simulink model "heli_q8_Lab3_primary"  (R2020b)
settings: Solver=ode1  StartTime=0.0  StopTime=inf  FixedStep=0.002  RelTol=1e-3  EnableMultiTasking=on
PostLoadFcn:
  | qc_set_target_type(getConfigSet(bdroot, 'QUARC Default Target Configuration'));
values from neighbouring files (symbols this model uses):
  A_lqr = [0, 1, 0, 0, 0 ... (first row only)    [init_heli_Lab3_extra.m]    (also in init_heli_Lab3_primary.m)
  B = [0 0; 0 K1; K2 0; 0 0; 0 0]    [init_heli_Lab3_extra.m]    (also in init_heli_Lab3_primary.m)
  C_lqr = [0 0 0 0 0 ... (first row only)    [init_heli_Lab3_extra.m]    (also in init_heli_Lab3_primary.m = [1 0 0 0 0)
  F = [0 0; 0 0]    [init_heli_Lab3_extra.m]    (also in init_heli_Lab3_primary.m = [1 0; 1 0])
  Joystick_gain_x = 1    [init_heli_Lab3_extra.m]    (also in init_heli_Lab3_primary.m)
  Joystick_gain_y = -1    [init_heli_Lab3_extra.m]    (also in init_heli_Lab3_primary.m)
  K_pd = -(lambda_1 + lambda_2)/K1    [init_heli_Lab3_extra.m]    (also in init_heli_Lab3_primary.m)
  K_pp = (lambda_1*lambda_2)/K1    [init_heli_Lab3_extra.m]    (also in init_heli_Lab3_primary.m)
  L = place(A_lqr', C_lqr', p).'    [init_heli_Lab3_extra.m]    (also in init_heli_Lab3_primary.m)
undefined symbols (not defined in the file or in its folder): HIL, K, qc_get_step_size
libraries: quarc_library x9
settings Model: SimulationMode=external  ExtModeTrigDuration=5000  Creator=Rchan  LastModifiedBy=pederaho
settings SolverCC: PositivePriorityOrder=on
settings DataIOCC: LimitDataPoints=on  SaveFormat=Array  SignalLoggingSaveFormat=ModelDataLogs  ReturnWorkspaceOutputs=off
settings OptimizationCC: ExpressionDepthLimit=2147483647  InitFltsAndDblsToZero=on  LifeSpan=inf
settings DebuggingCC: SaveWithParameterizedLinksMsg=none  UnderspecifiedInitializationDetection=Classic  MergeDetectMultiDrivingBlocksExec=none  SolverPrmCheckMsg=warning  MultiTaskDSMMsg=warning  MultiTaskCondExecSysMsg=none  FcnCallInpInsideContextMsg=warning  AllowSymbolicDim=off  StateNameClashWarn=warning  SFUnexpectedBacktrackingDiag=warning  SFNoUnconditionalDefaultTransitionDiag=warning  SFExecutionAtInitializationDiag=none  ArithmeticOperatorsInVariantConditions=warning
settings HardwareCC: ProdBitPerPointer=32  ProdBitPerSizeT=32  ProdBitPerPtrDiffT=32  ProdLargestAtomicFloat=None  ProdIntDivRoundTo=Undefined  ProdEndianess=Unspecified  ProdWordSize=32  ProdHWDeviceType=32-bit Generic
settings ModelReferenceCC: PropagateSignalLabelsOutOfModel=off
settings SFSimCC: SimUseLocalCustomCode=off  CustomCodeUndefinedFunction=UseInterfaceOnly
settings RTWCC: Description=QUARC Win64 Target  SystemTargetFile=quarc_win64.tlc  TemplateMakefile=quarc_default_tmf  RTWUseLocalCustomCode=off
settings CodeAppCC: StateflowObjectComments=on
settings GRTTargetCC: TargetLangStandard=C89/C90 (ANSI)  ParMdlRefBuildCompliant=off  CompOptLevelCompliant=off  CombineOutputUpdateFcns=off  MatFileLogging=off  GRTInterface=on  UseToolchainInfoCompliant=off  ExtMode=on  ExtModeMexFile=quarc_comm
settings ConfigComp: CovMetricSettings=dw  CovSaveCumulativeToWorkspaceVar=on  CovSaveSingleToWorkspaceVar=on  CovExternalEMLEnable=off  CovSFcnEnable=off

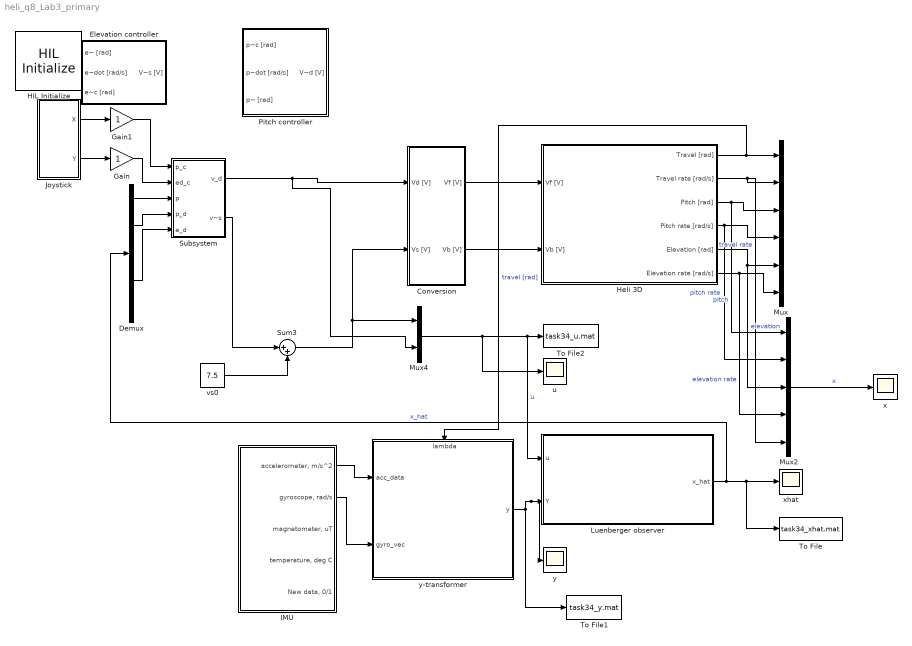
== system heli_q8_Lab3_primary ==
  Conversion : Subsystem
  Demux : Demux  Outputs=5
  Elevation controller : Subsystem
  Gain : Gain
  Gain1 : Gain
  HIL Initialize : quarc_library/Data Acquisition/Generic/Configuration/HIL Initialize  Priority=-99  object_name=HIL-1  board_type=q8_usb  board_number=0  board_options=update_rate=normal;decimation=1  exclusive=off  active=off  hardware_clocks=[0:2]  clock_modes=[]  initial_clock_frequencies=[]  set_clock_params_at_start=off  set_clock_params_at_switch_in=off  set_clock_frequencies_at_start=off  set_clock_frequencies_at_switch_in=off  analog_input_channels=[0:7]  analog_input_configurations=[]  analog_input_maximums=10  analog_input_minimums=-10  set_analog_input_params_at_start=on  set_analog_input_params_at_switch_in=off  analog_output_channels=[0:7]  analog_output_maximums=10  analog_output_minimums=-10  initial_analog_outputs=[0]  final_analog_outputs=[0]  watchdog_analog_outputs=0  set_analog_output_params_at_start=on  set_analog_output_params_at_switch_in=off  set_analog_outputs_at_start=on  set_analog_outputs_at_switch_in=off  set_analog_outputs_at_terminate=on  set_analog_outputs_at_switch_out=off  set_analog_outputs_on_watchdog=off  digital_input_channels=[]  digital_output_channels=[]  digital_output_configuration=[]  initial_digital_outputs=[1]  final_digital_outputs=[1]  watchdog_digital_outputs=[1]  set_digital_output_params_at_start=off  set_digital_output_params_at_switch_in=off  set_digital_outputs_at_start=on  set_digital_outputs_at_switch_in=off  set_digital_outputs_at_terminate=on  set_digital_outputs_at_switch_out=off  set_digital_outputs_on_watchdog=off  encoder_channels=[0:7]  quadrature=[4]  encoder_filter_frequency=[]  initial_encoder_counts=[0]  set_encoder_params_at_start=on  set_encoder_params_at_switch_in=off  set_encoder_counts_at_start=on  set_encoder_counts_at_switch_in=off  pwm_channels=[0:7]  pwm_modes=0  pwm_frequency=99.532799999999995e6/4095  pwm_configuration=[0]  pwm_alignment=[0]  pwm_polarity=[1]  pwm_leading_deadband=[0]  pwm_trailing_deadband=[0]  initial_pwm_outputs=[0]  final_pwm_outputs=[0]  watchdog_pwm_outputs=[0]  set_pwm_params_at_start=on  set_pwm_params_at_switch_in=off  set_pwm_outputs_at_start=on  set_pwm_outputs_at_switch_in=off  set_pwm_outputs_at_terminate=on  set_pwm_outputs_at_switch_out=off  set_pwm_outputs_on_watchdog=off  other_output_channels=[]  initial_other_outputs=[]  final_other_outputs=[]  watchdog_other_outputs=[]  set_other_outputs_at_start=off  set_other_outputs_at_switch_in=off  set_other_outputs_at_terminate=off  set_other_outputs_at_switch_out=off  set_other_outputs_on_watchdog=off
  Heli 3D : Subsystem
  IMU : Subsystem
  Joystick : Subsystem
  Luenberger observer : Subsystem
  Mux : Mux  Inputs=6
  Mux2 : Mux  Inputs=5
  Mux4 : Mux  Inputs=2
  Pitch controller : Subsystem
  Subsystem : Subsystem
  Sum3 : Sum  Inputs=|++
  To File : ToFile  Filename=task34_xhat.mat
  To File1 : ToFile  Filename=task34_y.mat
  To File2 : ToFile  Filename=task34_u.mat
  u : Scope
  vs0 : Constant  Value=7.5
  x : Scope
  xhat : Scope
  y : Scope
  y-transformer : Subsystem
      settings: PortSchema="{\"entries\":[{\"content\":{\"sides\":[{\"content\":{\"connectorIds\":[\"In1\",\"In2\"]},\"type\":\"ConnectorPlacement.EquallySpacedRectSide\",\"uuid\":\"7fe3842c-12da-4414-9d6c-fe9db8df7207\"},{\"content\":{\"connectorIds\":[\"Out1\"],\"side\":\"RIGHT\"},\"type\":\"ConnectorPlacement.EquallySpacedRectSide\",\"uuid\":\"81ab8372-6ad3-4160-a082-397e448f1dbf\"},{\"content\":{\"connectorIds\":[\"In3\"],\"side\":\"TOP\"},\"type\":\"ConnectorPlacement.EquallySpacedRectSide\",\"uuid\":\"eccdd19c-8bf4-44ad-b1cc-041d97ac8cb4\"},{\"content\":{\"connectorIds\":[],\"side\":\"HIDDEN\"},\"type\":\"ConnectorPlacement.EquallySpacedRectSide\",\"uuid\":\"e5e0ccf8-496d-4101-9f4c-362465ae7577\"}]},\"type\":\"ConnectorPlacement.EquallySpacedConnector\",\"uuid\":\"e1e81078-5ff0-43da-8bd4-b4064180551e\"}],\"packageUris\":[\"http://schema.mathworks.com/mf0/Connector/R2020b\"],\"version\":\"1.0\"}"
  wires:
  Mux2/1 -> x/1  "x"
  IMU/1("accelerometer, m/s^2") -> y-transformer/1(acc_data)
  Gain1/1 -> Subsystem/1(p_c)
  vs0/1 -> Sum3/2
  Subsystem/1(v_d) -> Mux4/2, Conversion/1(Vd [V])
  Demux/1 -> Subsystem/3(p)
  Sum3/1 -> Mux4/1, Conversion/2(Vs [V])
  Demux/2 -> Subsystem/4(p_d)
  Demux/4 -> Subsystem/5(e_d)
  Subsystem/2(v~s) -> Sum3/1
  IMU/2("gyroscope, rad/s") -> y-transformer/2(gyro_vec)
  Gain/1 -> Subsystem/2(ed_c)
  Joystick/2(Y) -> Gain/1
  Heli 3D/3(Pitch [rad]) -> Mux/3, Mux2/1  "pitch"
  Joystick/1(X) -> Gain1/1
  Heli 3D/1(Travel [rad]) -> Mux/1, y-transformer/3(lambda)  "travel [rad]"
  Conversion/1(Vf [V]) -> Heli 3D/1(Vf [V])
  Heli 3D/5(Elevation [rad]) -> Mux/5, Mux2/3  "elevation"
  Heli 3D/6(Elevation rate [rad/s]) -> Mux/6, Mux2/4  "elevation rate"
  Conversion/2(Vb [V]) -> Heli 3D/2(Vb [V])
  Luenberger observer/1(x_hat) -> xhat/1, To File/1, Demux/1  "x_hat"
  y-transformer/1(y) -> y/1, Luenberger observer/2(Y), To File1/1
  Mux4/1 -> Luenberger observer/1(u), To File2/1, u/1  "u"
  Heli 3D/2(Travel rate [rad/s]) -> Mux/2, Mux2/5  "travel rate"
  Heli 3D/4(Pitch rate [rad/s]) -> Mux/4, Mux2/2  "pitch rate"

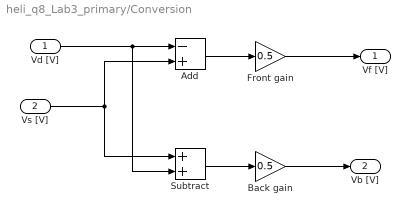
== system heli_q8_Lab3_primary/Conversion ==
  Vd [V] : Inport
  Vs [V] : Inport  Port=2
  Add : Sum  Inputs=-+
  Back gain : Gain  Gain=0.5
  Front gain : Gain  Gain=0.5
  Subtract : Sum
  Vf [V] : Outport
  Vb [V] : Outport  Port=2
  wires:
  Vd [V]/1 -> Subtract/2, Add/1
  Vs [V]/1 -> Subtract/1, Add/2
  Subtract/1 -> Back gain/1
  Back gain/1 -> Vb [V]/1
  Add/1 -> Front gain/1
  Front gain/1 -> Vf [V]/1

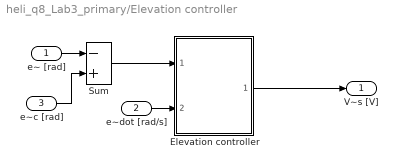
== system heli_q8_Lab3_primary/Elevation controller ==
  e~ [rad] : Inport
  e~dot [rad/s] : Inport  Port=2
  e~c [rad] : Inport  Port=3
  Elevation controller : Subsystem
  Sum : Sum  Inputs=-+  InputSameDT=on  SaturateOnIntegerOverflow=on  OutDataTypeStr=Inherit: Same as first input
  V~s [V] : Outport  InitialOutput=0
  wires:
  Sum/1 -> Elevation controller/1(e~ [rad])
  Elevation controller/1(V~_s [V]) -> V~s [V]/1
  e~ [rad]/1 -> Sum/1
  e~dot [rad/s]/1 -> Elevation controller/2(e~_dot [rad/s])
  e~c [rad]/1 -> Sum/2

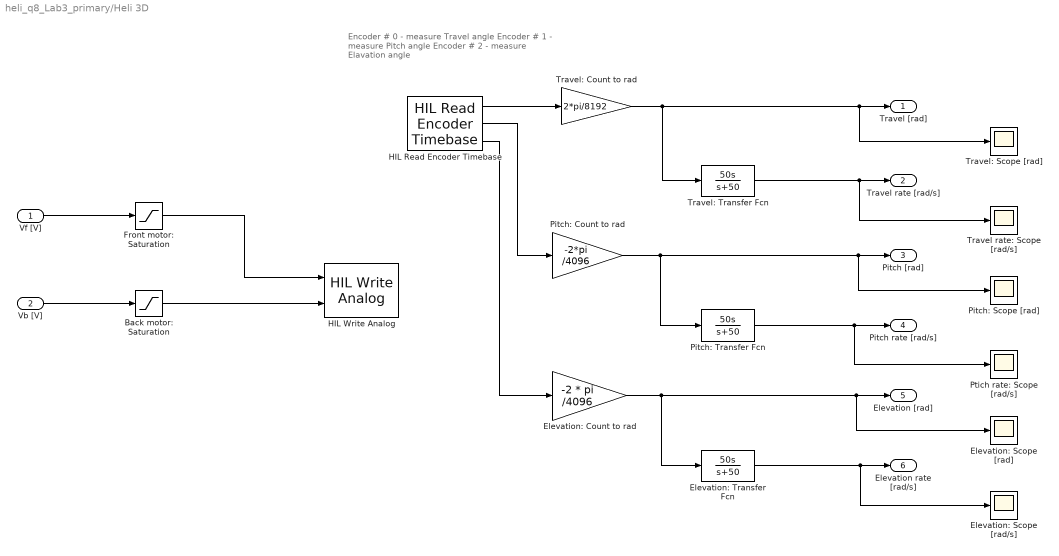
== system heli_q8_Lab3_primary/Heli 3D ==
  note: Encoder # 0 - measure Travel angle
      | Encoder # 1 - measure Pitch angle
      | Encoder # 2 - measure Elavation angle
  Vf [V] : Inport
  Vb [V] : Inport  Port=2
  Back motor: Saturation : Saturate  UpperLimit=5  LowerLimit=-5
  Elevation: Count to rad : Gain  Gain=-2 * pi /4096
  Elevation: Scope [rad/s] : Scope
  Elevation: Scope [rad] : Scope
  Elevation: Transfer Fcn : TransferFcn  Numerator=[50 0]  Denominator=[1 50]
  Front motor: Saturation : Saturate  UpperLimit=5  LowerLimit=-5
  HIL Read Encoder Timebase : quarc_library/Data Acquisition/Generic/Timebases/HIL Read Encoder Timebase  object_name=HIL-1  clock=0  channels=[0:2]  active=on  vector_output=off  data_type_mode=Inherit via back propagation  data_type=double  overflow_mode=Error on overflow  samples_in_buffer=max(ceil(1/qc_get_step_size), 1)
  HIL Write Analog : quarc_library/Data Acquisition/Generic/Immediate I//O/HIL Write Analog  object_name=HIL-1  channels=[0:1]  sample_time=-1  active=off  vector_input=off
  Pitch: Count to rad : Gain  Gain=-2*pi /4096
  Pitch: Scope [rad] : Scope
  Pitch: Transfer Fcn : TransferFcn  Numerator=[50 0]  Denominator=[1 50]
  Ptich rate: Scope [rad/s] : Scope
  Travel rate: Scope [rad/s] : Scope
  Travel: Count to rad : Gain  Gain=2*pi/8192
  Travel: Scope [rad] : Scope
  Travel: Transfer Fcn : TransferFcn  Numerator=[50 0]  Denominator=[1 50]
  Travel [rad] : Outport
  Travel rate [rad/s] : Outport  Port=2
  Pitch [rad] : Outport  Port=3
  Pitch rate [rad/s] : Outport  Port=4
  Elevation [rad] : Outport  Port=5
  Elevation rate [rad/s] : Outport  Port=6
  wires:
  HIL Read Encoder Timebase/1 -> Travel: Count to rad/1
  HIL Read Encoder Timebase/2 -> Pitch: Count to rad/1
  HIL Read Encoder Timebase/3 -> Elevation: Count to rad/1
  Travel: Count to rad/1 -> Travel: Scope [rad]/1, Travel [rad]/1, Travel: Transfer Fcn/1
  Travel: Transfer Fcn/1 -> Travel rate: Scope [rad/s]/1, Travel rate [rad/s]/1
  Pitch: Count to rad/1 -> Pitch: Transfer Fcn/1, Pitch: Scope [rad]/1, Pitch [rad]/1
  Pitch: Transfer Fcn/1 -> Ptich rate: Scope [rad/s]/1, Pitch rate [rad/s]/1
  Elevation: Count to rad/1 -> Elevation: Transfer Fcn/1, Elevation: Scope [rad]/1, Elevation [rad]/1
  Elevation: Transfer Fcn/1 -> Elevation: Scope [rad/s]/1, Elevation rate [rad/s]/1
  Vf [V]/1 -> Front motor: Saturation/1
  Vb [V]/1 -> Back motor: Saturation/1
  Front motor: Saturation/1 -> HIL Write Analog/1
  Back motor: Saturation/1 -> HIL Write Analog/2

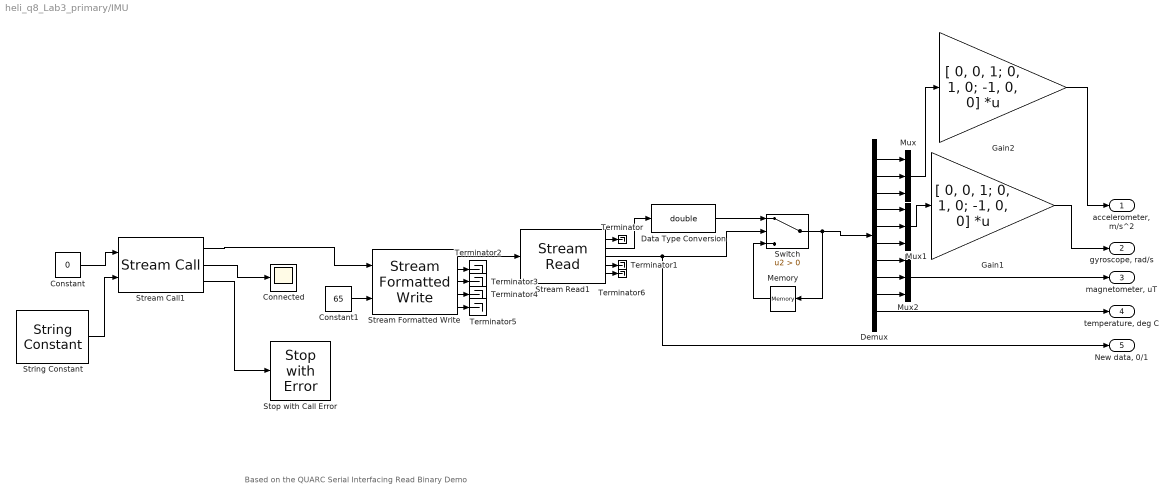
== system heli_q8_Lab3_primary/IMU ==
  note: Based on the QUARC Serial Interfacing Read Binary Demo
  Connected : Scope
  Constant : Constant  Value=0
  Constant1 : Constant  Value=65
  Data Type Conversion : DataTypeConversion  OutDataTypeStr=double
  Demux : Demux  Outputs=10
  Gain1 : Gain  Gain=[ 0, 0, 1; 0, 1, 0; -1, 0, 0]  Multiplication=Matrix(K*u) (u vector)
  Gain2 : Gain  Gain=[ 0, 0, 1; 0, 1, 0; -1, 0, 0]  Multiplication=Matrix(K*u) (u vector)
  Memory : Memory  InitialCondition=[0 0 0 0 0 0 0 0 0 0]
  Mux : Mux  Inputs=3
  Mux1 : Mux  Inputs=3
  Mux2 : Mux  Inputs=3
  Stop with Call Error : quarc_library/Sinks/Error Handling/Stop with Error  message_type=Interpret input as error code  message=Error occurred
      settings: SourceProductName=QUARC Targets
  Stream Call1 : quarc_library/Communications/Intermediate/Stream Call  uri_source=External input port  uri=serial://IMU:9?baud=115200,word=8,parity=none,stop=1,flow='none'  apply_uri_to_all_configs=on  send_buffer_size=8000  receive_buffer_size=8000  byte_order=little endian (Intel - LSB first)  sample_time=qc_get_step_size  non_blocking=on  active=off
      settings: SourceProductName=QUARC Targets
  Stream Formatted Write : quarc_library/Communications/Intermediate/Stream Formatted Write  format_string=%c\n  max_code_units=80  optimization=Minimizing latency
      settings: SourceProductName=QUARC Targets
  Stream Read1 : quarc_library/Communications/Intermediate/Stream Read  data_type=single  type_expr=BusObject  num_elements=10  receive_dims=off
      settings: SourceProductName=QUARC Targets
  String Constant : quarc_library/Strings/String Constant  string_value=qc_perform_substitutions('serial://IMU:%{PORT}?baud=115200,word=8,parity=none,stop=1')  evaluate_string=on  string_type=URI  max_length=255  sample_time=inf  variable_size=off
      settings: AttributesFormatString="\"serial://IMU:4?baud=115200,word=8,parity=none,stop=1\""  SourceProductName=QUARC Targets
  Switch : Switch  Criteria=u2 > Threshold
  Terminator{,1..6} (7 alike) : Terminator
  "accelerometer, m/s^2" : Outport
  "gyroscope, rad/s" : Outport  Port=2
  "magnetometer, uT" : Outport  Port=3
  "temperature, deg C" : Outport  Port=4
  "New data, 0/1" : Outport  Port=5
  wires:
  Switch/1 -> Memory/1, Demux/1
  Data Type Conversion/1 -> Switch/1
  Stream Read1/3 -> "New data, 0/1"/1, Switch/2
  Stream Formatted Write/1 -> Stream Read1/1
  Constant1/1 -> Stream Formatted Write/2
  Gain1/1 -> "gyroscope, rad/s"/1
  Gain2/1 -> "accelerometer, m/s^2"/1
  Stream Read1/4 -> Terminator1/1
  Demux/10 -> "temperature, deg C"/1
  Mux1/1 -> Gain1/1
  Stream Read1/2 -> Data Type Conversion/1
  Demux/7 -> Mux2/1
  Demux/8 -> Mux2/2
  Demux/9 -> Mux2/3
  Mux2/1 -> "magnetometer, uT"/1
  Demux/6 -> Mux1/3
  Demux/5 -> Mux1/2
  Demux/4 -> Mux1/1
  Mux/1 -> Gain2/1
  Demux/3 -> Mux/3
  Demux/1 -> Mux/1
  Demux/2 -> Mux/2
  Stream Read1/1 -> Terminator/1
  Stream Call1/1 -> Stream Formatted Write/1
  Constant/1 -> Stream Call1/1
  String Constant/1 -> Stream Call1/2
  Stream Call1/2 -> Connected/1
  Stream Call1/3 -> Stop with Call Error/1
  Memory/1 -> Switch/3
  Stream Formatted Write/2 -> Terminator2/1
  Stream Formatted Write/3 -> Terminator3/1
  Stream Formatted Write/4 -> Terminator4/1
  Stream Formatted Write/5 -> Terminator5/1
  Stream Read1/5 -> Terminator6/1

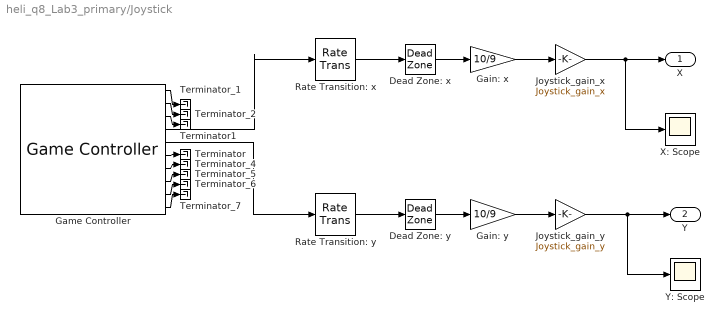
== system heli_q8_Lab3_primary/Joystick ==
  Dead Zone: x : DeadZone  LowerValue=-0.1  UpperValue=0.1  SaturateOnIntegerOverflow=on
  Dead Zone: y : DeadZone  LowerValue=-0.1  UpperValue=0.1  SaturateOnIntegerOverflow=on
  Gain: x : Gain  Gain=10/9
  Gain: y : Gain  Gain=10/9
  Game Controller : quarc_library/Devices/Peripherals/Target/Game Controller  controller=1  buffer_size=12  deadzone=[]  saturation=[]  sample_time=max(qc_get_step_size, 0.01)  auto_center=off  enabled=on
      settings: SourceProductName=QUARC Targets
  Joystick_gain_x : Gain  Gain=Joystick_gain_x
  Joystick_gain_y : Gain  Gain=Joystick_gain_y
  Rate Transition: x : RateTransition
  Rate Transition: y : RateTransition
  Terminator : Terminator
  Terminator1 : Terminator
  Terminator_{1..2,4..7} (6 alike) : Terminator
  X: Scope : Scope
  Y: Scope : Scope
  X : Outport
  Y : Outport  Port=2
  wires:
  Rate Transition: y/1 -> Dead Zone: y/1
  Rate Transition: x/1 -> Dead Zone: x/1
  Game Controller/5 -> Rate Transition: y/1
  Game Controller/4 -> Rate Transition: x/1
  Game Controller/1 -> Terminator_1/1
  Game Controller/2 -> Terminator_2/1
  Game Controller/7 -> Terminator_4/1
  Game Controller/8 -> Terminator_5/1
  Game Controller/9 -> Terminator_6/1
  Game Controller/10 -> Terminator_7/1
  Game Controller/3 -> Terminator1/1
  Game Controller/6 -> Terminator/1
  Dead Zone: x/1 -> Gain: x/1
  Dead Zone: y/1 -> Gain: y/1
  Gain: x/1 -> Joystick_gain_x/1
  Gain: y/1 -> Joystick_gain_y/1
  Joystick_gain_x/1 -> X/1, X: Scope/1
  Joystick_gain_y/1 -> Y: Scope/1, Y/1

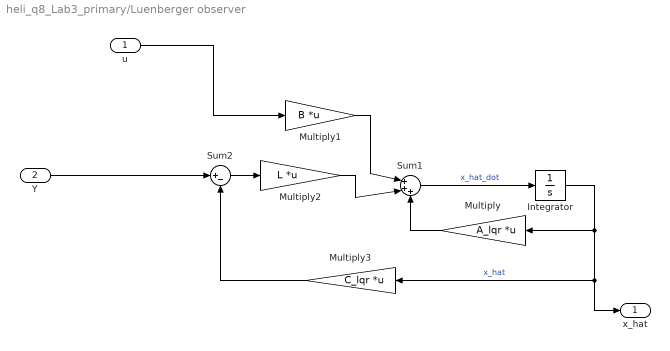
== system heli_q8_Lab3_primary/Luenberger observer ==
  u : Inport
  Y : Inport  Port=2
  Integrator : Integrator
  Multiply : Gain  Gain=A_lqr  Multiplication=Matrix(K*u) (u vector)
  Multiply1 : Gain  Gain=B  Multiplication=Matrix(K*u) (u vector)
  Multiply2 : Gain  Gain=L  Multiplication=Matrix(K*u) (u vector)
  Multiply3 : Gain  Gain=C_lqr  Multiplication=Matrix(K*u) (u vector)
  Sum1 : Sum  Inputs=|+++
  Sum2 : Sum  Inputs=|+-
  x_hat : Outport
  wires:
  Multiply/1 -> Sum1/3
  Multiply2/1 -> Sum1/2
  Multiply1/1 -> Sum1/1
  Integrator/1 -> x_hat/1, Multiply3/1, Multiply/1  "x_hat"
  Sum2/1 -> Multiply2/1
  u/1 -> Multiply1/1
  Multiply3/1 -> Sum2/2
  Sum1/1 -> Integrator/1  "x_hat_dot"
  Y/1 -> Sum2/1

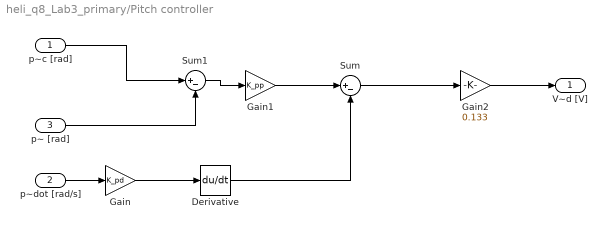
== system heli_q8_Lab3_primary/Pitch controller ==
  p~c [rad] : Inport
  p~dot [rad/s] : Inport  Port=2
  p~ [rad] : Inport  Port=3
  Derivative : Derivative
  Gain : Gain  Gain=K_pd
  Gain1 : Gain  Gain=K_pp
  Gain2 : Gain  Gain=0.133
  Sum : Sum  Inputs=|+-
  Sum1 : Sum  Inputs=|+-
  V~d [V] : Outport  InitialOutput=0
  wires:
  p~dot [rad/s]/1 -> Gain/1
  Gain/1 -> Derivative/1
  Derivative/1 -> Sum/2
  p~c [rad]/1 -> Sum1/1
  p~ [rad]/1 -> Sum1/2
  Sum1/1 -> Gain1/1
  Gain1/1 -> Sum/1
  Sum/1 -> Gain2/1
  Gain2/1 -> V~d [V]/1

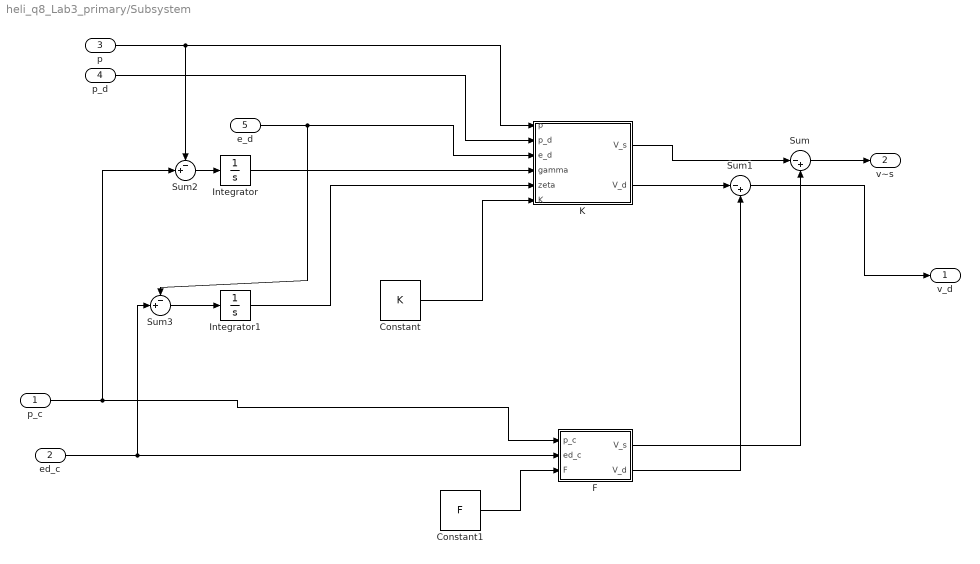
== system heli_q8_Lab3_primary/Subsystem ==
  p_c : Inport
  ed_c : Inport  Port=2
  p : Inport  Port=3
  p_d : Inport  Port=4
  e_d : Inport  Port=5
  Constant : Constant  Value=K
  Constant1 : Constant  Value=F
  F : MATLAB Function  TreatAsAtomicUnit=on
  Integrator : Integrator
  Integrator1 : Integrator
  K : MATLAB Function  TreatAsAtomicUnit=on
  Sum : Sum  Inputs=|-+
  Sum1 : Sum  Inputs=|-+
  Sum2 : Sum  Inputs=-+|
  Sum3 : Sum  Inputs=-+|
  v_d : Outport
  v~s : Outport  Port=2
  wires:
  p/1 -> Sum2/1, K/1(p)
  p_d/1 -> K/2(p_d)
  e_d/1 -> Sum3/1, K/3(e_d)
  Constant/1 -> K/6(K)
  Constant1/1 -> F/3(F)
  p_c/1 -> Sum2/2, F/1(p_c)
  ed_c/1 -> Sum3/2, F/2(ed_c)
  K/1(V_s) -> Sum/1
  Sum/1 -> v~s/1
  K/2(V_d) -> Sum1/1
  F/1(V_s) -> Sum/2
  F/2(V_d) -> Sum1/2
  Sum1/1 -> v_d/1
  Integrator/1 -> K/4(gamma)
  Integrator1/1 -> K/5(zeta)
  Sum2/1 -> Integrator/1
  Sum3/1 -> Integrator1/1

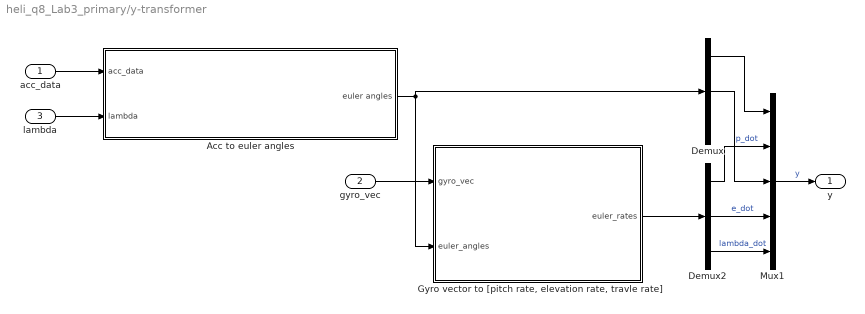
== system heli_q8_Lab3_primary/y-transformer ==
  acc_data : Inport
  gyro_vec : Inport  Port=2
  lambda : Inport  Port=3
  Acc to euler angles : Subsystem
  Demux : Demux  Outputs=3
  Demux2 : Demux  Outputs=3
  "Gyro vector to [pitch rate, elevation rate, travle rate]" : MATLAB Function  TreatAsAtomicUnit=on
  Mux1 : Mux  Inputs=5
  y : Outport
  wires:
  acc_data/1 -> Acc to euler angles/1(acc_data)
  "Gyro vector to [pitch rate, elevation rate, travle rate]"/1(euler_rates) -> Demux2/1
  Demux/2 -> Mux1/3
  Demux/1 -> Mux1/1
  Demux2/2 -> Mux1/4  "e_dot"
  Demux2/1 -> Mux1/2  "p_dot"
  gyro_vec/1 -> "Gyro vector to [pitch rate, elevation rate, travle rate]"/1(gyro_vec)
  Demux2/3 -> Mux1/5  "lambda_dot"
  Mux1/1 -> y/1  "y"
  Acc to euler angles/1(euler angles) -> Demux/1, "Gyro vector to [pitch rate, elevation rate, travle rate]"/2(euler_angles)
  lambda/1 -> Acc to euler angles/2(lambda)

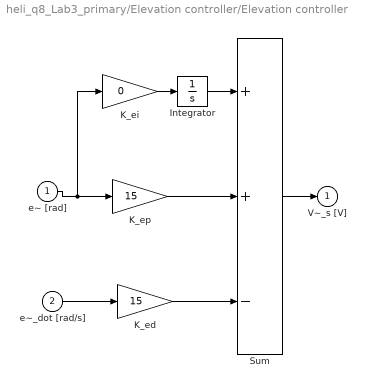
== system heli_q8_Lab3_primary/Elevation controller/Elevation controller ==
  e~ [rad] : Inport
  e~_dot [rad/s] : Inport  Port=2
  Integrator : Integrator  LimitOutput=on
  K_ed : Gain  Gain=15  SaturateOnIntegerOverflow=on  OutDataTypeStr=Inherit: Same as input  ParamDataTypeStr=Inherit: Same as input
  K_ei : Gain  Gain=0  SaturateOnIntegerOverflow=on  OutDataTypeStr=Inherit: Same as input  ParamDataTypeStr=Inherit: Same as input
  K_ep : Gain  Gain=15  SaturateOnIntegerOverflow=on  OutDataTypeStr=Inherit: Same as input  ParamDataTypeStr=Inherit: Same as input
  Sum : Sum  Inputs=++-  InputSameDT=on  SaturateOnIntegerOverflow=on  OutDataTypeStr=Inherit: Same as first input
  V~_s [V] : Outport  InitialOutput=0
  wires:
  K_ei/1 -> Integrator/1
  Integrator/1 -> Sum/1
  Sum/1 -> V~_s [V]/1
  e~_dot [rad/s]/1 -> K_ed/1
  K_ed/1 -> Sum/3
  K_ep/1 -> Sum/2
  e~ [rad]/1 -> K_ep/1, K_ei/1

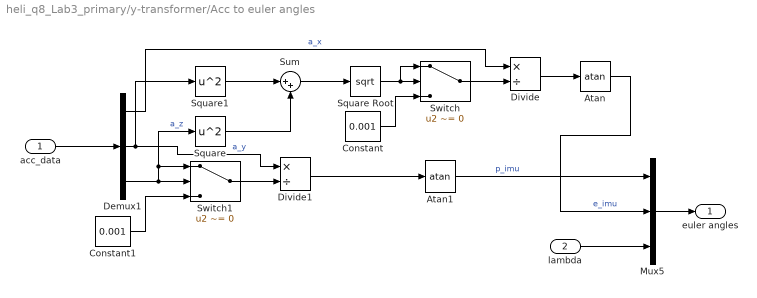
== system heli_q8_Lab3_primary/y-transformer/Acc to euler angles ==
  acc_data : Inport
  lambda : Inport  Port=2
  Atan : Trigonometry  Operator=atan
  Atan1 : Trigonometry  Operator=atan
  Constant : Constant  Value=0.001
  Constant1 : Constant  Value=0.001
  Demux1 : Demux  Outputs=3
  Divide : Product  Inputs=*/  RndMeth=Zero  SaturateOnIntegerOverflow=on
  Divide1 : Product  Inputs=*/  RndMeth=Zero  SaturateOnIntegerOverflow=on
  Mux5 : Mux  Inputs=3
  Square : Math  Operator=square  SaturateOnIntegerOverflow=on
  Square Root : Sqrt  SaturateOnIntegerOverflow=on
  Square1 : Math  Operator=square  SaturateOnIntegerOverflow=on
  Sum : Sum  Inputs=|++
  Switch : Switch  Criteria=u2 ~= 0
  Switch1 : Switch  Criteria=u2 ~= 0
  euler angles : Outport
  wires:
  acc_data/1 -> Demux1/1
  lambda/1 -> Mux5/3
  Sum/1 -> Square Root/1
  Constant1/1 -> Switch1/3
  Square/1 -> Sum/2
  Atan1/1 -> Mux5/1  "p_imu"
  Square Root/1 -> Switch/1, Switch/2
  Square1/1 -> Sum/1
  Constant/1 -> Switch/3
  Switch1/1 -> Divide1/2
  Divide/1 -> Atan/1
  Switch/1 -> Divide/2
  Atan/1 -> Mux5/2  "e_imu"
  Divide1/1 -> Atan1/1
  Demux1/1 -> Divide/1  "a_x"
  Mux5/1 -> euler angles/1
  Demux1/3 -> Switch1/1, Square/1, Switch1/2  "a_z"
  Demux1/2 -> Divide1/1, Square1/1  "a_y"

== matlab function heli_q8_Lab3_primary/Subsystem/F ==
  data: p_c input; V_s output; V_d output; ed_c input; F input
function [V_s, V_d] = fcn(p_c, ed_c, F)
M = (F*[p_c, ed_c].');
V_s = M(1, :);
V_d = M(2, :);
end

== matlab function heli_q8_Lab3_primary/Subsystem/K ==
  data: p input; V_s output; V_d output; p_d input; e_d input; gamma input; zeta input; K input
function [V_s, V_d] = fcn(p, p_d, e_d, gamma, zeta, K)
M = (K*[p, p_d, e_d, gamma, zeta].');
V_s = M(1, :);
V_d = M(2, :);
end

== matlab function heli_q8_Lab3_primary/y-transformer/Gyro vector to [pitch rate, elevation rate, travle rate] ==
  data: gyro_vec input; euler_rates output; euler_angles input
function euler_rates = gyro_vec_to_euler_rates(gyro_vec,euler_angles)
%#codegen
    phi = euler_angles(1);
    theta = euler_angles(2);
    %psi = euler_angles(3);


    T = [1, sin(phi)*tan(theta), cos(phi)*tan(theta);
         0, cos(phi),            -sin(phi);
         0, sin(phi)/cos(theta), cos(phi)/cos(theta)]; 
euler_rates = T*gyro_vec;
